simulink model "Sistema"  (R2026b)
settings: Solver=ode15s  StopTime=15  MaxStep=1E-2
libraries: fl_lib x6, nesl_utility x3, slpidlib x2, ee_lib x1
settings Model: Creator=HP  LastModifiedBy=19ram
settings DataIOCC: DSMLogging=off  ReturnWorkspaceOutputs=off  SaveOutput=off  SignalLogging=off  TimeSaveName=t
settings DebuggingCC: AlgebraicLoopMsg=none  ArtificialAlgebraicLoopMsg=none  MaxConsecutiveZCsMsg=none
settings SimscapeCC: SimscapeLogType=all  SimscapeNominalValues="[{\"value\":\"1\",\"unit\":\"A\"},{\"value\":\"1\",\"unit\":\"bar\"},{\"value\":\"1\",\"unit\":\"cm^2\"},{\"value\":\"1\",\"unit\":\"cm^3/s\"},{\"value\":\"1\",\"unit\":\"kJ/kg\"},{\"value\":\"1\",\"unit\":\"kW\"},{\"value\":\"1\",\"unit\":\"l\"},{\"value\":\"1\",\"unit\":\"N\"},{\"value\":\"1\",\"unit\":\"N*m\"},{\"value\":\"1\",\"unit\":\"V\"},{\"value\":\"0.001\",\"unit\":\"Wb\"}]"  SimscapeUseEnergyAccounting=off

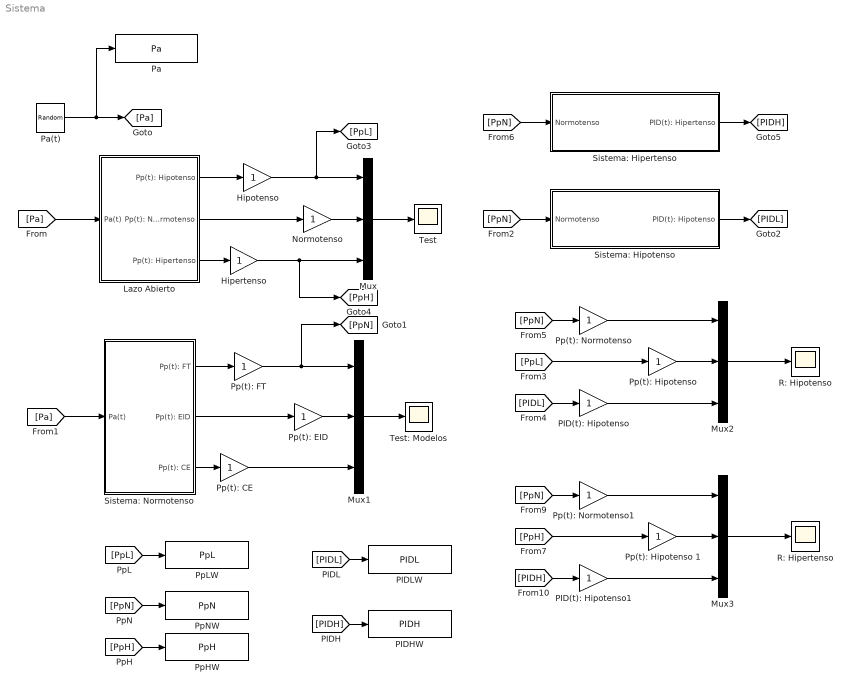
== system Sistema ==
  Hipertenso : Gain
  Hipotenso : Gain
  Lazo Abierto : Subsystem
  Mux{,1..3} (4 alike) : Mux  Inputs=3
  Normotenso : Gain
  PID(t): Hipotenso : Gain
  PID(t): Hipotenso1 : Gain
  PIDHW : ToWorkspace  VariableName=PIDH  SampleTime=-1
  PIDLW : ToWorkspace  VariableName=PIDL  SampleTime=-1
  Pa : ToWorkspace  VariableName=Pa  SampleTime=-1
  Pa(t) : UniformRandomNumber  Minimum=-0.2  Seed=106  SampleTime=0.1
  Pp(t): CE : Gain
  Pp(t): EID : Gain
  Pp(t): FT : Gain
  "Pp(t): Hipotenso " : Gain
  Pp(t): Hipotenso 1 : Gain
  Pp(t): Normotenso : Gain
  Pp(t): Normotenso1 : Gain
  PpHW : ToWorkspace  VariableName=PpH  SampleTime=-1
  PpLW : ToWorkspace  VariableName=PpL  SampleTime=-1
  PpNW : ToWorkspace  VariableName=PpN  SampleTime=-1
  R: Hipertenso : Scope
      settings: ActiveDisplayYMinimum=-0.534843699383776  ActiveDisplayYMaximum=1.3457713865770577  YLabel=V(t)  DataLoggingVariableName=ScopeData3
  R: Hipotenso : Scope
      settings: ActiveDisplayYMinimum=-0.534843699383776  ActiveDisplayYMaximum=1.3457713865770577  YLabel=V(t)  DataLoggingVariableName=ScopeData2
  Sistema: Hipertenso : Subsystem
  Sistema: Hipotenso : Subsystem
  Sistema: Normotenso : Subsystem
  Test : Scope
      settings: ActiveDisplayYMinimum=-0.534843699383776  ActiveDisplayYMaximum=1.3457713865770577  YLabel=V(t)
  Test: Modelos : Scope
      settings: ActiveDisplayYMinimum=-0.534843699383776  ActiveDisplayYMaximum=1.3457713865770577  YLabel=V(t)
  wires:
  Lazo Abierto/2(Pp(t): Normotenso) -> Normotenso/1
  Lazo Abierto/1(Pp(t): Hipotenso) -> Hipotenso/1
  Lazo Abierto/3(Pp(t): Hipertenso) -> Hipertenso/1
  Pa(t)/1 -> Pa/1, [Pa]
  [Pa] -> Lazo Abierto/1(Pa(t))
  Mux/1 -> Test/1
  Hipotenso/1 -> [PpL], Mux/1
  Normotenso/1 -> Mux/2
  Hipertenso/1 -> [PpH], Mux/3
  [Pa] -> Sistema: Normotenso/1(Pa(t))
  Pp(t): CE/1 -> Mux1/3
  Pp(t): EID/1 -> Mux1/2
  Pp(t): FT/1 -> [PpN], Mux1/1
  Mux1/1 -> Test: Modelos/1
  Sistema: Normotenso/1(Pp(t): FT) -> Pp(t): FT/1
  Sistema: Normotenso/2(Pp(t): EID) -> Pp(t): EID/1
  Sistema: Normotenso/3(Pp(t): CE) -> Pp(t): CE/1
  [PpN] -> Sistema: Hipotenso/1(Normotenso)
  Sistema: Hipotenso/1(PID(t): Hipotenso) -> [PIDL]
  [PIDL] -> PID(t): Hipotenso/1
  [PpL] -> "Pp(t): Hipotenso "/1
  [PpN] -> Pp(t): Normotenso/1
  Mux2/1 -> R: Hipotenso/1
  Pp(t): Normotenso/1 -> Mux2/1
  "Pp(t): Hipotenso "/1 -> Mux2/2
  PID(t): Hipotenso/1 -> Mux2/3
  [PpN] -> Sistema: Hipertenso/1(Normotenso)
  Sistema: Hipertenso/1(PID(t): Hipertenso) -> [PIDH]
  Mux3/1 -> R: Hipertenso/1
  Pp(t): Normotenso1/1 -> Mux3/1
  [PpH] -> Pp(t): Hipotenso 1/1
  [PpN] -> Pp(t): Normotenso1/1
  [PIDH] -> PID(t): Hipotenso1/1
  PID(t): Hipotenso1/1 -> Mux3/3
  Pp(t): Hipotenso 1/1 -> Mux3/2
  [PpH] -> PpHW/1
  [PpN] -> PpNW/1
  [PpL] -> PpLW/1
  [PIDL] -> PIDLW/1
  [PIDH] -> PIDHW/1

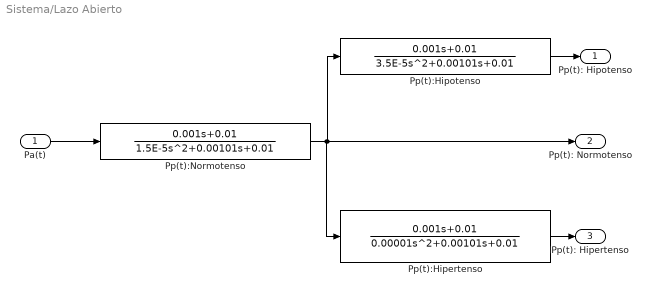
== system Sistema/Lazo Abierto ==
  Pa(t) : Inport
  Pp(t):Hipertenso : TransferFcn  Numerator=[0.001,0.01]  Denominator=[0.00001,0.00101,0.01]
  Pp(t):Hipotenso : TransferFcn  Numerator=[0.001,0.01]  Denominator=[3.5E-5,0.00101,0.01]
  Pp(t):Normotenso : TransferFcn  Numerator=[0.001,0.01]  Denominator=[1.5E-5,0.00101,0.01]
  Pp(t): Hipotenso : Outport
  Pp(t): Normotenso : Outport  Port=2
  Pp(t): Hipertenso : Outport  Port=3
  wires:
  Pa(t)/1 -> Pp(t):Normotenso/1
  Pp(t):Hipotenso/1 -> Pp(t): Hipotenso/1
  Pp(t):Normotenso/1 -> Pp(t):Hipertenso/1, Pp(t):Hipotenso/1, Pp(t): Normotenso/1
  Pp(t):Hipertenso/1 -> Pp(t): Hipertenso/1

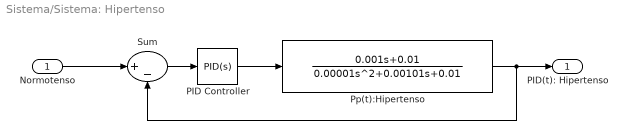
== system Sistema/Sistema: Hipertenso ==
  Normotenso : Inport
  PID Controller : slpidlib/PID Controller  Controller=PID  Form=Parallel  TimeDomain=Continuous-time  UseExternalTs=off  SampleTime=-1  IntegratorMethod=Forward Euler  FilterMethod=Forward Euler  ControllerParametersSource=internal  P=129.9786  I=312762.8587  UseKiTs=off  D=0.0017461  UseExternalDerivativeSource=off  N=49610.1327  UseFilter=on  TunerSelectOption=Transfer Function Based (PID Tuner App)  InitialConditionSource=internal  InitialConditionForIntegrator=0  InitialConditionForFilter=0  DifferentiatorICPrevScaledInput=0  ExternalReset=none  TrackingMode=off  Kt=1  LimitOutput=off  SatLimitsSource=internal  UpperSaturationLimit=inf  LowerSaturationLimit=-inf  LinearizeAsGain=on  AntiWindupMode=none  Kb=1  LimitIntegrator=off  UpperIntegratorSaturationLimit=inf  LowerIntegratorSaturationLimit=-inf  POutMin=[]  POutMax=[]  IOutMin=[]  IOutMax=[]  DOutMin=[]  DOutMax=[]  NOutMin=[]  NOutMax=[]  SumOutMin=[]  SumOutMax=[]  SaturationOutMin=[]  SaturationOutMax=[]  PParamMin=[]  PParamMax=[]  IParamMin=[]  IParamMax=[]  DParamMin=[]  DParamMax=[]  NParamMin=[]  NParamMax=[]  KbParamMin=[]  KbParamMax=[]  KtParamMin=[]  KtParamMax=[]  KbOutMin=[]  KbOutMax=[]  KtOutMin=[]  KtOutMax=[]  IntegratorOutMin=[]  IntegratorOutMax=[]  FilterOutMin=[]  FilterOutMax=[]  SumI1OutMin=[]  SumI1OutMax=[]  SumI2OutMin=[]  SumI2OutMax=[]  SumI3OutMin=[]  SumI3OutMax=[]  SumI4OutMin=[]  SumI4OutMax=[]  SumDOutMin=[]  SumDOutMax=[]  DifferentiatorOutMin=[]  DifferentiatorOutMax=[]  FilterDiffOutCoefMin=[]  FilterDiffOutCoefMax=[]  ReciprocalOutMin=[]  ReciprocalOutMax=[]  SumDenOutMin=[]  SumDenOutMax=[]  SumNumOutMin=[]  SumNumOutMax=[]  DivideOutMin=[]  DivideOutMax=[]  UdiffTsProdOutMin=[]  UdiffTsProdOutMax=[]  NTsProdOutMin=[]  NTsProdOutMax=[]  UintegralTsProdOutMin=[]  UintegralTsProdOutMax=[]  UngainTsProdOutMin=[]  UngainTsProdOutMax=[]  ClampingZeroOutDataTypeStr=Inherit: Inherit via back propagation  ClampingZeroOutMin=[]  ClampingZeroOutMax=[]  FilterDenConstantOutDataTypeStr=Inherit: Inherit via back propagation  FilterDenConstantOutMin=[]  FilterDenConstantOutMax=[]  PCopyOutDataTypeStr=Inherit: Inherit via back propagation  PCopyOutMin=[]  PCopyOutMax=[]  NCopyOutDataTypeStr=Inherit: Inherit via back propagation  NCopyOutMin=[]  NCopyOutMax=[]  IntegratorContinuousStateAttributes=''  IntegratorStateMustResolveToSignalObject=off  IntegratorRTWStateStorageClass=Auto  FilterContinuousStateAttributes=''  FilterStateMustResolveToSignalObject=off  FilterRTWStateStorageClass=Auto  ParallelPVariant=InternalParameters  IdealPVariant=Disabled  IVariant=InternalParameters  DVariant=InternalParameters  IntegratorVariant=Continuous  SatVariant=Disabled  AWVariant=Passthrough  PCopyVariant=Disabled  TRVariant=Disabled  FdbkBlocksVariant=Forward  IdealPFdbkVariant=Disabled  SatFdbkVariant=Disabled  DerivativeFilterVariant=ContFilter  NVariant=InternalParameters  NCopyVariant=Disabled  FilterICVariant=InternalICsFilter  IntegratorICVariant=InternalICs  ExternalResetVariant=Disabled  TRSumVariant=Passthrough  SumFdbkVariant=Disabled  SumVariant=Sum_PID  TsampFilterVariant=InternalTs  TsampNgainVariant=Passthrough  TsampIntegralVariant=Disabled_SignalSpec  ExternalSaturationOutDataTypeStr=Inherit: Same as second input  DerivativeSourceVariant=ErrorSignal  PreIntVariant=InternalPreInt
  Pp(t):Hipertenso : TransferFcn  Numerator=[0.001,0.01]  Denominator=[0.00001,0.00101,0.01]
  Sum : Sum  Inputs=|+-
  PID(t): Hipertenso : Outport
  wires:
  PID Controller/1 -> Pp(t):Hipertenso/1
  Normotenso/1 -> Sum/1
  Sum/1 -> PID Controller/1
  Pp(t):Hipertenso/1 -> Sum/2, PID(t): Hipertenso/1

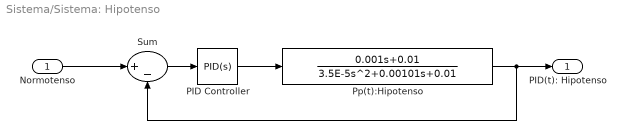
== system Sistema/Sistema: Hipotenso ==
  Normotenso : Inport
  PID Controller : slpidlib/PID Controller  Controller=PID  Form=Parallel  TimeDomain=Continuous-time  UseExternalTs=off  SampleTime=-1  IntegratorMethod=Forward Euler  FilterMethod=Forward Euler  ControllerParametersSource=internal  P=458.48258315116  I=1112094.73550687  UseKiTs=off  D=0.00626713168710677  UseExternalDerivativeSource=off  N=50057.6250783319  UseFilter=on  TunerSelectOption=Transfer Function Based (PID Tuner App)  InitialConditionSource=internal  InitialConditionForIntegrator=0  InitialConditionForFilter=0  DifferentiatorICPrevScaledInput=0  ExternalReset=none  TrackingMode=off  Kt=1  LimitOutput=off  SatLimitsSource=internal  UpperSaturationLimit=inf  LowerSaturationLimit=-inf  LinearizeAsGain=on  AntiWindupMode=none  Kb=1  LimitIntegrator=off  UpperIntegratorSaturationLimit=inf  LowerIntegratorSaturationLimit=-inf  POutMin=[]  POutMax=[]  IOutMin=[]  IOutMax=[]  DOutMin=[]  DOutMax=[]  NOutMin=[]  NOutMax=[]  SumOutMin=[]  SumOutMax=[]  SaturationOutMin=[]  SaturationOutMax=[]  PParamMin=[]  PParamMax=[]  IParamMin=[]  IParamMax=[]  DParamMin=[]  DParamMax=[]  NParamMin=[]  NParamMax=[]  KbParamMin=[]  KbParamMax=[]  KtParamMin=[]  KtParamMax=[]  KbOutMin=[]  KbOutMax=[]  KtOutMin=[]  KtOutMax=[]  IntegratorOutMin=[]  IntegratorOutMax=[]  FilterOutMin=[]  FilterOutMax=[]  SumI1OutMin=[]  SumI1OutMax=[]  SumI2OutMin=[]  SumI2OutMax=[]  SumI3OutMin=[]  SumI3OutMax=[]  SumI4OutMin=[]  SumI4OutMax=[]  SumDOutMin=[]  SumDOutMax=[]  DifferentiatorOutMin=[]  DifferentiatorOutMax=[]  FilterDiffOutCoefMin=[]  FilterDiffOutCoefMax=[]  ReciprocalOutMin=[]  ReciprocalOutMax=[]  SumDenOutMin=[]  SumDenOutMax=[]  SumNumOutMin=[]  SumNumOutMax=[]  DivideOutMin=[]  DivideOutMax=[]  UdiffTsProdOutMin=[]  UdiffTsProdOutMax=[]  NTsProdOutMin=[]  NTsProdOutMax=[]  UintegralTsProdOutMin=[]  UintegralTsProdOutMax=[]  UngainTsProdOutMin=[]  UngainTsProdOutMax=[]  ClampingZeroOutDataTypeStr=Inherit: Inherit via back propagation  ClampingZeroOutMin=[]  ClampingZeroOutMax=[]  FilterDenConstantOutDataTypeStr=Inherit: Inherit via back propagation  FilterDenConstantOutMin=[]  FilterDenConstantOutMax=[]  PCopyOutDataTypeStr=Inherit: Inherit via back propagation  PCopyOutMin=[]  PCopyOutMax=[]  NCopyOutDataTypeStr=Inherit: Inherit via back propagation  NCopyOutMin=[]  NCopyOutMax=[]  IntegratorContinuousStateAttributes=''  IntegratorStateMustResolveToSignalObject=off  IntegratorRTWStateStorageClass=Auto  FilterContinuousStateAttributes=''  FilterStateMustResolveToSignalObject=off  FilterRTWStateStorageClass=Auto  ParallelPVariant=InternalParameters  IdealPVariant=Disabled  IVariant=InternalParameters  DVariant=InternalParameters  IntegratorVariant=Continuous  SatVariant=Disabled  AWVariant=Passthrough  PCopyVariant=Disabled  TRVariant=Disabled  FdbkBlocksVariant=Forward  IdealPFdbkVariant=Disabled  SatFdbkVariant=Disabled  DerivativeFilterVariant=ContFilter  NVariant=InternalParameters  NCopyVariant=Disabled  FilterICVariant=InternalICsFilter  IntegratorICVariant=InternalICs  ExternalResetVariant=Disabled  TRSumVariant=Passthrough  SumFdbkVariant=Disabled  SumVariant=Sum_PID  TsampFilterVariant=InternalTs  TsampNgainVariant=Passthrough  TsampIntegralVariant=Disabled_SignalSpec  ExternalSaturationOutDataTypeStr=Inherit: Same as second input  DerivativeSourceVariant=ErrorSignal  PreIntVariant=InternalPreInt
  Pp(t):Hipotenso : TransferFcn  Numerator=[0.001,0.01]  Denominator=[3.5E-5,0.00101,0.01]
  Sum : Sum  Inputs=|+-
  PID(t): Hipotenso : Outport
  wires:
  PID Controller/1 -> Pp(t):Hipotenso/1
  Normotenso/1 -> Sum/1
  Sum/1 -> PID Controller/1
  Pp(t):Hipotenso/1 -> Sum/2, PID(t): Hipotenso/1

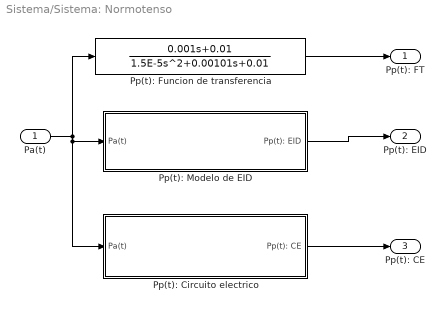
== system Sistema/Sistema: Normotenso ==
  Pa(t) : Inport
  Pp(t): Circuito electrico : Subsystem
  Pp(t): Funcion de transferencia : TransferFcn  Numerator=[0.001,0.01]  Denominator=[1.5E-5,0.00101,0.01]
  Pp(t): Modelo de EID : Subsystem
  Pp(t): FT : Outport
  Pp(t): EID : Outport  Port=2
  Pp(t): CE : Outport  Port=3
  wires:
  Pa(t)/1 -> Pp(t): Circuito electrico/1(Pa(t)), Pp(t): Modelo de EID/1(Pa(t)), Pp(t): Funcion de transferencia/1
  Pp(t): Funcion de transferencia/1 -> Pp(t): FT/1
  Pp(t): Modelo de EID/1(Pp(t): EID) -> Pp(t): EID/1
  Pp(t): Circuito electrico/1(Pp(t): CE) -> Pp(t): CE/1

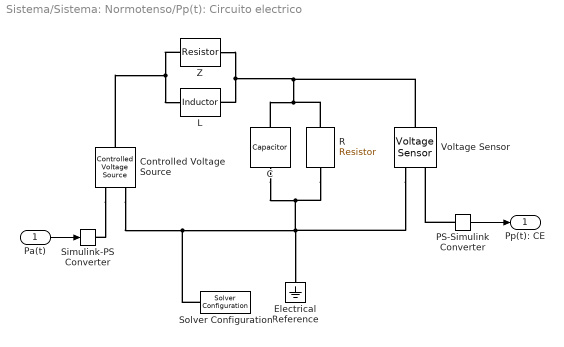
== system Sistema/Sistema: Normotenso/Pp(t): Circuito electrico ==
  Pa(t) : Inport
  C : fl_lib/Electrical/Electrical Elements/Capacitor  c=1.5 F  r=1e-6 Ohm  g=0 1/Ohm  i_specify=off  i_priority=None  i=0 A  i_nominal_specify=off  i_nominal_value=1  i_nominal_unit=A  v_specify=off  v_priority=None  v=0 V  v_nominal_specify=off  v_nominal_value=1  v_nominal_unit=V  vc_specify=off  vc_priority=High  vc=0 V  vc_nominal_specify=off  vc_nominal_value=1  vc_nominal_unit=V
  Controlled Voltage Source : fl_lib/Electrical/Electrical Sources/Controlled Voltage Source
  Electrical Reference : fl_lib/Electrical/Electrical Elements/Electrical Reference
  L : ee_lib/Passive/Inductor  l=0.001 H  enable_L_tol=ee.enum.toleranceApplication.none  L_tol=20  tol_distribution=ee.enum.toleranceDistribution.uniform  nSigma=4  r=0 Ohm  g=1e-9 1/Ohm  enable_operating_limits=ee.enum.enable.no  operating_limit_action=ee.enum.passive.reportOpLim.warn  max_working_current=1 A  power_rating=1 W  i_L_specify=off  i_L_priority=High  i_L=0 A  i_L_nominal_specify=off  i_L_nominal_value=1  i_L_nominal_unit=A
  PS-Simulink Converter : nesl_utility/PS-Simulink Converter  PhysicalDomain=network_engine_domain  SubClassName=ps_output  LeftPortType=input  RightPortType=output  PseudoPeriodic=off  Frequencies=[]  VectorFormat=inherit  Unit=inherit  AffineConversion=off
  R : fl_lib/Electrical/Electrical Elements/Resistor  R=1 Ohm  i_specify=off  i_priority=None  i=0 A  i_nominal_specify=off  i_nominal_value=1  i_nominal_unit=A  v_specify=off  v_priority=None  v=0 V  v_nominal_specify=off  v_nominal_value=1  v_nominal_unit=V
  Simulink-PS Converter : nesl_utility/Simulink-PS Converter  PhysicalDomain=network_engine_domain  SubClassName=ps_input  LeftPortType=input  RightPortType=output  PseudoPeriodic=off  Frequencies=[]  NoiseDistribution=none  NoiseParameters=[]  Unit=1  AffineConversion=off  FilteringAndDerivatives=provide  SimscapeFilterOrder=1  InputFilterTimeConstant=0.001  UdotUserProvided=0
  Solver Configuration : nesl_utility/Solver Configuration  PhysicalDomain=network_engine_domain  SubClassName=solver  LeftPortType=input  RightPortType=generic  Tones=[]  Harmonics=[]  SimulateNoise=off  Profile=off  UseLocalSampling=off  EnableSwitchedLinearOptims=on  FrequencyDomain=off  UseCCode=off  RelTol=0.001  AbsTol=0.001  MinStep=1e-09  ToWorkspace=off  RevertToSquareIcSolve=off  NumHomotopyIterations=100  PhasorMode=off  PhasorModeNumHarmonics=1  ConsistencySolver=NEWTON_XTOL_AFTER_FTOL  CanonicalOrdering=CANONICAL  OptimizeIntermediates=OPTIMIZED  MulticoreSolverChoice=BACKWARD_EULER  IndexReductionMethod=DerivativeReplacement  DoDC=off  ResidualTolerance=1e-09  ConsistencyTolSource=GLOBAL  ConsistencyAbsTol=0.001  ConsistencyRelTol=0.001  ConsistencyTolFactor=0.001  UseLocalSolver=off  LocalSolverChoice=NE_BACKWARD_EULER_ADVANCER  ResolveIndetEquations=on  FunctionEvalNumThread=1  LocalSolverSampleTime=0.001  DoFixedCost=off  MaxNonlinIter=3  MaxModeIter=2  ComputeImpulses=off  ImpulseIterations=2  LinearAlgebra=auto  LinearAlgebraNumThread=0  EquationFormulation=NE_TIME_EF  DelaysMemoryBudget=1024  AutomaticFiltering=on  FilteringTimeConstant=0.001  PartitionStorageMethod=AS_NEEDED  PartitionMemoryBudget=1024  PartitionMethod=BALANCED  MultibodyUseLocalSolver=off  MultibodyLocalSolverChoice=ODE1  MultibodyLocalSolverSampleTime=0.001
  Voltage Sensor : fl_lib/Electrical/Electrical Sensors/Voltage Sensor
  Z : fl_lib/Electrical/Electrical Elements/Resistor  R=0.010 Ohm  i_specify=off  i_priority=None  i=0 A  i_nominal_specify=off  i_nominal_value=1  i_nominal_unit=A  v_specify=off  v_priority=None  v=0 V  v_nominal_specify=off  v_nominal_value=1  v_nominal_unit=V
  Pp(t): CE : Outport
  wires:
  Pa(t)/1 -> Simulink-PS Converter/1
  PS-Simulink Converter/1 -> Pp(t): CE/1
  connections:
  Z/LConn1 -- Controlled Voltage Source/LConn1 -- L/LConn1
  C/LConn1 -- Voltage Sensor/LConn1 -- Z/RConn1 -- L/RConn1 -- R/LConn1
  Controlled Voltage Source/RConn1 -- Simulink-PS Converter/RConn1
  Controlled Voltage Source/RConn2 -- Solver Configuration/RConn1 -- Voltage Sensor/RConn2 -- R/RConn1 -- C/RConn1 -- Electrical Reference/LConn1
  PS-Simulink Converter/LConn1 -- Voltage Sensor/RConn1

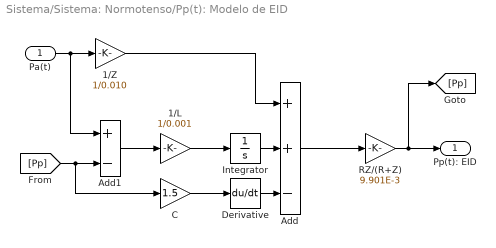
== system Sistema/Sistema: Normotenso/Pp(t): Modelo de EID ==
  Pa(t) : Inport
  1/L : Gain  Gain=1/0.001
  1/Z : Gain  Gain=1/0.010
  Add : Sum  Inputs=++-
  Add1 : Sum  Inputs=+-
  C : Gain  Gain=1.5
  Derivative : Derivative
  Integrator : Integrator
  RZ/(R+Z) : Gain  Gain=9.901E-3
  Pp(t): EID : Outport
  wires:
  Add/1 -> RZ/(R+Z)/1
  RZ/(R+Z)/1 -> [Pp], Pp(t): EID/1
  1/Z/1 -> Add/1
  Pa(t)/1 -> 1/Z/1, Add1/1
  [Pp] -> C/1, Add1/2
  Add1/1 -> 1/L/1
  Integrator/1 -> Add/2
  1/L/1 -> Integrator/1
  Derivative/1 -> Add/3
  C/1 -> Derivative/1
